simulink model "Inverter_32Vrms_StaticFreq_Fixed"  (R2025b)
settings: Solver=FixedStepDiscrete  StartTime=0.0  StopTime=0.35  FixedStep=SPWM_Ts  RelTol=1e-3
InitFcn:
  | evalin(get_param('Inverter_32Vrms_StaticFreq_Fixed','ModelWorkspace'),'assert(isscalar(SPWM_f1) && isfinite(SPWM_f1) && SPWM_f1>=20 && SPWM_f1<=100, ''SPWM_f1 must be 20 to 100 Hz.''); CL_N=round(1/(SPWM_f1*CL_Ts)); CL_AA_a=exp(-2*pi*CL_faa*SPWM_Ts); CL_AAComp=((1-CL_AA_a)^2+2*CL_AA_a*(1-cos(2*pi*SPWM_f1*SPWM_Ts)))/(1-CL_AA_a)^2;');
model workspace (MAT data in the model file):
  CL_AAComp = 1.00999999872
  CL_AA_a = 0.998744152176
  CL_Kaw = 20
  CL_Ki = 1.2
  CL_Kp = 0.02
  CL_N = 100
  CL_Ts = 0.0001
  CL_Vref = 32
  CL_faa = 1000
  CL_fp = 50
  CL_mff = 0.95
  CL_mmax = 1
  SPWM_Ndead = 10
  SPWM_Tdead = 2e-06
  SPWM_Ts = 2e-07
  SPWM_Vgate = 10
  SPWM_f1 = 100
  SPWM_fs = 20000
  SPWM_m = 0.8
undefined symbols (not defined in the file): DiscIntNeverNeededParam
libraries: fl_lib x19, ee_lib x13, nesl_utility x13
settings Model: Creator=liuhaobo  LastModifiedBy=liuhaobo

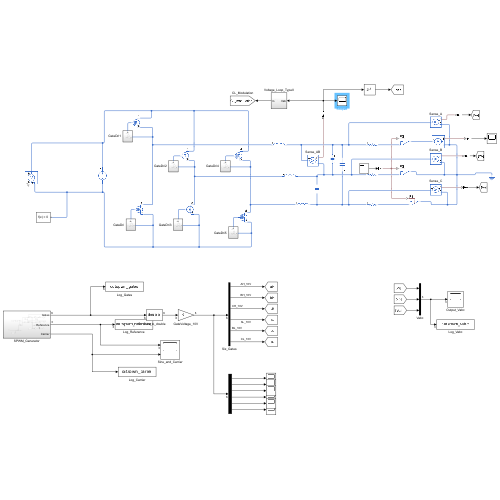
[thumbnail: Simulink's stored preview of the top-level diagram]
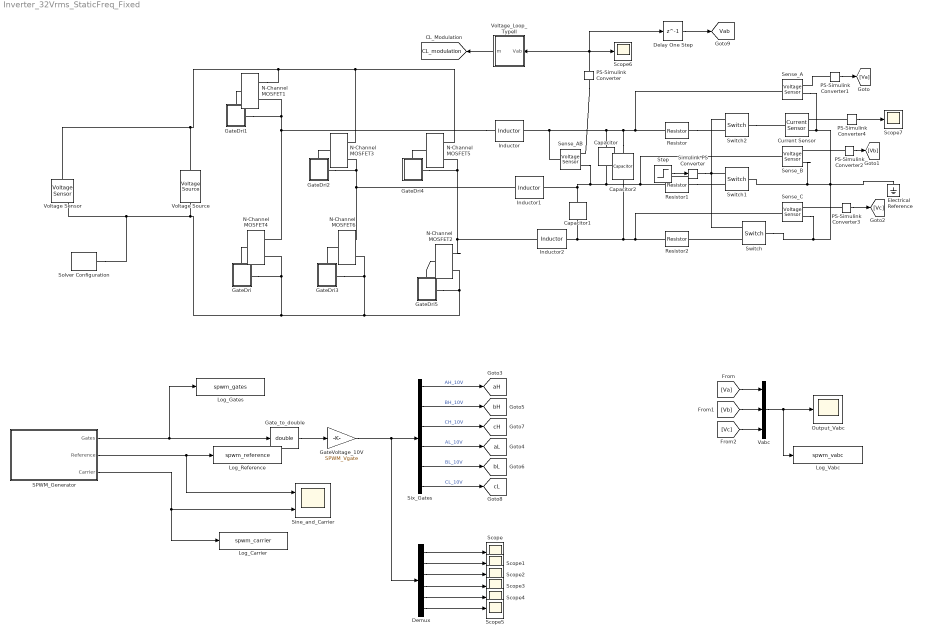
== system Inverter_32Vrms_StaticFreq_Fixed ==
  Capacitor : ee_lib/Passive/Capacitor  cap_option=ee.enum.passive.capacitor.capOption.const  c=2 uF  Cvec=[1e-05, 1e-06] F  Vvec=[0, 10] V  CV_table_symmetry=ee.enum.passive.capacitor.tableSymmetry.yes  f_vec=[1, 10] kHz  DFext_vec=[.8, 1.2]  enable_C_tol=ee.enum.toleranceApplication.none  averaging_period=0 s  C_tol=5  tol_distribution=ee.enum.toleranceDistribution.uniform  nSigma=4  r=0 Ohm  g=0 1/Ohm  enable_operating_limits=ee.enum.enable.no  operating_limit_action=ee.enum.passive.reportOpLim.warn  max_working_voltage_range=[-25, 25] V  power_rating=1 W  maxTemperature=85 degC  thermalEnable=false  thermalMass=1 J/K  i_specify=off  i_priority=None  i=0 A  i_nominal_specify=off  i_nominal_value=1  i_nominal_unit=A  v_specify=off  v_priority=None  v=0 V  v_nominal_specify=off  v_nominal_value=1  v_nominal_unit=V  vc_specify=off  vc_priority=High  vc=0 V  vc_nominal_specify=off  vc_nominal_value=1  vc_nominal_unit=V  T_specify=off  T_priority=None  T=298.15 K  T_nominal_specify=off  T_nominal_value=1  T_nominal_unit=K
  Capacitor1 : ee_lib/Passive/Capacitor  cap_option=ee.enum.passive.capacitor.capOption.const  c=2 uF  Cvec=[1e-05, 1e-06] F  Vvec=[0, 10] V  CV_table_symmetry=ee.enum.passive.capacitor.tableSymmetry.yes  f_vec=[1, 10] kHz  DFext_vec=[.8, 1.2]  enable_C_tol=ee.enum.toleranceApplication.none  averaging_period=0 s  C_tol=5  tol_distribution=ee.enum.toleranceDistribution.uniform  nSigma=4  r=0 Ohm  g=0 1/Ohm  enable_operating_limits=ee.enum.enable.no  operating_limit_action=ee.enum.passive.reportOpLim.warn  max_working_voltage_range=[-25, 25] V  power_rating=1 W  maxTemperature=85 degC  thermalEnable=false  thermalMass=1 J/K  i_specify=off  i_priority=None  i=0 A  i_nominal_specify=off  i_nominal_value=1  i_nominal_unit=A  v_specify=off  v_priority=None  v=0 V  v_nominal_specify=off  v_nominal_value=1  v_nominal_unit=V  vc_specify=off  vc_priority=High  vc=0 V  vc_nominal_specify=off  vc_nominal_value=1  vc_nominal_unit=V  T_specify=off  T_priority=None  T=298.15 K  T_nominal_specify=off  T_nominal_value=1  T_nominal_unit=K
  Capacitor2 : ee_lib/Passive/Capacitor  cap_option=ee.enum.passive.capacitor.capOption.const  c=2 uF  Cvec=[1e-05, 1e-06] F  Vvec=[0, 10] V  CV_table_symmetry=ee.enum.passive.capacitor.tableSymmetry.yes  f_vec=[1, 10] kHz  DFext_vec=[.8, 1.2]  enable_C_tol=ee.enum.toleranceApplication.none  averaging_period=0 s  C_tol=5  tol_distribution=ee.enum.toleranceDistribution.uniform  nSigma=4  r=0 Ohm  g=0 1/Ohm  enable_operating_limits=ee.enum.enable.no  operating_limit_action=ee.enum.passive.reportOpLim.warn  max_working_voltage_range=[-25, 25] V  power_rating=1 W  maxTemperature=85 degC  thermalEnable=false  thermalMass=1 J/K  i_specify=off  i_priority=None  i=0 A  i_nominal_specify=off  i_nominal_value=1  i_nominal_unit=A  v_specify=off  v_priority=None  v=0 V  v_nominal_specify=off  v_nominal_value=1  v_nominal_unit=V  vc_specify=off  vc_priority=High  vc=0 V  vc_nominal_specify=off  vc_nominal_value=1  vc_nominal_unit=V  T_specify=off  T_priority=None  T=298.15 K  T_nominal_specify=off  T_nominal_value=1  T_nominal_unit=K
  Current Sensor : fl_lib/Electrical/Electrical Sensors/Current Sensor
  Delay One Step : Delay  DelayLength=1
  Demux : Demux  Outputs=6
  Electrical Reference : fl_lib/Electrical/Electrical Elements/Electrical Reference
  GateDri : Subsystem
      settings: PortSchema="{\"entries\":[{\"content\":{\"sides\":[{\"content\":{\"connectorIds\":[\"LConn1\"]},\"type\":\"ConnectorPlacement.EquallySpacedRectSide\",\"uuid\":\"5ec2b66a-2e5f-4a29-ad7d-11e5a28469f4\"},{\"content\":{\"side\":\"RIGHT\"},\"type\":\"ConnectorPlacement.EquallySpacedRectSide\",\"uuid\":\"968cf12b-ade8-46ac-9f94-1e8ea2f3f677\"},{\"content\":{\"side\":\"TOP\"},\"type\":\"ConnectorPlacement.EquallySpacedRectSide\",\"uuid\":\"41030f6a-5ac0-4230-aa4b-0c03378f97d6\"},{\"content\":{\"connectorIds\":[\"RConn1\"],\"side\":\"BOTTOM\"},\"type\":\"ConnectorPlacement.EquallySpacedRectSide\",\"uuid\":\"8f964c8e-6f21-4ad0-8f7c-edbb0b22c660\"}]},\"type\":\"ConnectorPlacement.EquallySpacedConnector\",\"uuid\":\"dccfb76b-3882-476d-8e51-da801e2932e6\"}],\"packageUris\":[\"http://schema.mathworks.com/mf0/Connector/R2020b\"],\"version\":\"1.0\"}"
  GateDri1 : Subsystem
      settings: PortSchema="{\"entries\":[{\"content\":{\"sides\":[{\"content\":{\"connectorIds\":[\"LConn1\"]},\"type\":\"ConnectorPlacement.EquallySpacedRectSide\",\"uuid\":\"5ec2b66a-2e5f-4a29-ad7d-11e5a28469f4\"},{\"content\":{\"side\":\"RIGHT\"},\"type\":\"ConnectorPlacement.EquallySpacedRectSide\",\"uuid\":\"968cf12b-ade8-46ac-9f94-1e8ea2f3f677\"},{\"content\":{\"side\":\"TOP\"},\"type\":\"ConnectorPlacement.EquallySpacedRectSide\",\"uuid\":\"41030f6a-5ac0-4230-aa4b-0c03378f97d6\"},{\"content\":{\"connectorIds\":[\"RConn1\"],\"side\":\"BOTTOM\"},\"type\":\"ConnectorPlacement.EquallySpacedRectSide\",\"uuid\":\"8f964c8e-6f21-4ad0-8f7c-edbb0b22c660\"}]},\"type\":\"ConnectorPlacement.EquallySpacedConnector\",\"uuid\":\"dccfb76b-3882-476d-8e51-da801e2932e6\"}],\"packageUris\":[\"http://schema.mathworks.com/mf0/Connector/R2020b\"],\"version\":\"1.0\"}"
  GateDri2 : Subsystem
      settings: PortSchema="{\"entries\":[{\"content\":{\"sides\":[{\"content\":{\"connectorIds\":[\"LConn1\"]},\"type\":\"ConnectorPlacement.EquallySpacedRectSide\",\"uuid\":\"5ec2b66a-2e5f-4a29-ad7d-11e5a28469f4\"},{\"content\":{\"side\":\"RIGHT\"},\"type\":\"ConnectorPlacement.EquallySpacedRectSide\",\"uuid\":\"968cf12b-ade8-46ac-9f94-1e8ea2f3f677\"},{\"content\":{\"side\":\"TOP\"},\"type\":\"ConnectorPlacement.EquallySpacedRectSide\",\"uuid\":\"41030f6a-5ac0-4230-aa4b-0c03378f97d6\"},{\"content\":{\"connectorIds\":[\"RConn1\"],\"side\":\"BOTTOM\"},\"type\":\"ConnectorPlacement.EquallySpacedRectSide\",\"uuid\":\"8f964c8e-6f21-4ad0-8f7c-edbb0b22c660\"}]},\"type\":\"ConnectorPlacement.EquallySpacedConnector\",\"uuid\":\"dccfb76b-3882-476d-8e51-da801e2932e6\"}],\"packageUris\":[\"http://schema.mathworks.com/mf0/Connector/R2020b\"],\"version\":\"1.0\"}"
  GateDri3 : Subsystem
      settings: PortSchema="{\"entries\":[{\"content\":{\"sides\":[{\"content\":{\"connectorIds\":[\"LConn1\"]},\"type\":\"ConnectorPlacement.EquallySpacedRectSide\",\"uuid\":\"5ec2b66a-2e5f-4a29-ad7d-11e5a28469f4\"},{\"content\":{\"side\":\"RIGHT\"},\"type\":\"ConnectorPlacement.EquallySpacedRectSide\",\"uuid\":\"968cf12b-ade8-46ac-9f94-1e8ea2f3f677\"},{\"content\":{\"side\":\"TOP\"},\"type\":\"ConnectorPlacement.EquallySpacedRectSide\",\"uuid\":\"41030f6a-5ac0-4230-aa4b-0c03378f97d6\"},{\"content\":{\"connectorIds\":[\"RConn1\"],\"side\":\"BOTTOM\"},\"type\":\"ConnectorPlacement.EquallySpacedRectSide\",\"uuid\":\"8f964c8e-6f21-4ad0-8f7c-edbb0b22c660\"}]},\"type\":\"ConnectorPlacement.EquallySpacedConnector\",\"uuid\":\"dccfb76b-3882-476d-8e51-da801e2932e6\"}],\"packageUris\":[\"http://schema.mathworks.com/mf0/Connector/R2020b\"],\"version\":\"1.0\"}"
  GateDri4 : Subsystem
      settings: PortSchema="{\"entries\":[{\"content\":{\"sides\":[{\"content\":{\"connectorIds\":[\"LConn1\"]},\"type\":\"ConnectorPlacement.EquallySpacedRectSide\",\"uuid\":\"5ec2b66a-2e5f-4a29-ad7d-11e5a28469f4\"},{\"content\":{\"side\":\"RIGHT\"},\"type\":\"ConnectorPlacement.EquallySpacedRectSide\",\"uuid\":\"968cf12b-ade8-46ac-9f94-1e8ea2f3f677\"},{\"content\":{\"side\":\"TOP\"},\"type\":\"ConnectorPlacement.EquallySpacedRectSide\",\"uuid\":\"41030f6a-5ac0-4230-aa4b-0c03378f97d6\"},{\"content\":{\"connectorIds\":[\"RConn1\"],\"side\":\"BOTTOM\"},\"type\":\"ConnectorPlacement.EquallySpacedRectSide\",\"uuid\":\"8f964c8e-6f21-4ad0-8f7c-edbb0b22c660\"}]},\"type\":\"ConnectorPlacement.EquallySpacedConnector\",\"uuid\":\"dccfb76b-3882-476d-8e51-da801e2932e6\"}],\"packageUris\":[\"http://schema.mathworks.com/mf0/Connector/R2020b\"],\"version\":\"1.0\"}"
  GateDri5 : Subsystem
      settings: PortSchema="{\"entries\":[{\"content\":{\"sides\":[{\"content\":{\"connectorIds\":[\"LConn1\"]},\"type\":\"ConnectorPlacement.EquallySpacedRectSide\",\"uuid\":\"5ec2b66a-2e5f-4a29-ad7d-11e5a28469f4\"},{\"content\":{\"side\":\"RIGHT\"},\"type\":\"ConnectorPlacement.EquallySpacedRectSide\",\"uuid\":\"968cf12b-ade8-46ac-9f94-1e8ea2f3f677\"},{\"content\":{\"side\":\"TOP\"},\"type\":\"ConnectorPlacement.EquallySpacedRectSide\",\"uuid\":\"41030f6a-5ac0-4230-aa4b-0c03378f97d6\"},{\"content\":{\"connectorIds\":[\"RConn1\"],\"side\":\"BOTTOM\"},\"type\":\"ConnectorPlacement.EquallySpacedRectSide\",\"uuid\":\"8f964c8e-6f21-4ad0-8f7c-edbb0b22c660\"}]},\"type\":\"ConnectorPlacement.EquallySpacedConnector\",\"uuid\":\"dccfb76b-3882-476d-8e51-da801e2932e6\"}],\"packageUris\":[\"http://schema.mathworks.com/mf0/Connector/R2020b\"],\"version\":\"1.0\"}"
  GateVoltage_10V : Gain  Gain=SPWM_Vgate
  Gate_to_double : DataTypeConversion  OutDataTypeStr=double  SaturateOnIntegerOverflow=off  RndMeth=Floor
  Inductor : ee_lib/Passive/Inductor  l=680 uH  enable_L_tol=ee.enum.toleranceApplication.none  L_tol=20  tol_distribution=ee.enum.toleranceDistribution.uniform  nSigma=4  r=0 Ohm  g=1e-9 1/Ohm  enable_operating_limits=ee.enum.enable.no  operating_limit_action=ee.enum.passive.reportOpLim.warn  max_working_current=1 A  power_rating=1 W  i_L_specify=off  i_L_priority=High  i_L=0 A  i_L_nominal_specify=off  i_L_nominal_value=1  i_L_nominal_unit=A
  Inductor1 : ee_lib/Passive/Inductor  l=680 uH  enable_L_tol=ee.enum.toleranceApplication.none  L_tol=20  tol_distribution=ee.enum.toleranceDistribution.uniform  nSigma=4  r=0 Ohm  g=1e-9 1/Ohm  enable_operating_limits=ee.enum.enable.no  operating_limit_action=ee.enum.passive.reportOpLim.warn  max_working_current=1 A  power_rating=1 W  i_L_specify=off  i_L_priority=High  i_L=0 A  i_L_nominal_specify=off  i_L_nominal_value=1  i_L_nominal_unit=A
  Inductor2 : ee_lib/Passive/Inductor  l=680 uH  enable_L_tol=ee.enum.toleranceApplication.none  L_tol=20  tol_distribution=ee.enum.toleranceDistribution.uniform  nSigma=4  r=0 Ohm  g=1e-9 1/Ohm  enable_operating_limits=ee.enum.enable.no  operating_limit_action=ee.enum.passive.reportOpLim.warn  max_working_current=1 A  power_rating=1 W  i_L_specify=off  i_L_priority=High  i_L=0 A  i_L_nominal_specify=off  i_L_nominal_value=1  i_L_nominal_unit=A
  Log_Carrier : ToWorkspace  VariableName=spwm_carrier  SaveFormat=Timeseries  SampleTime=-1
  Log_Gates : ToWorkspace  VariableName=spwm_gates  SaveFormat=Timeseries  SampleTime=-1
  Log_Reference : ToWorkspace  VariableName=spwm_reference  SaveFormat=Timeseries  SampleTime=-1
  Log_Vabc : ToWorkspace  VariableName=spwm_vabc  SaveFormat=Timeseries  SampleTime=-1
  N-Channel MOSFET{1..6} (6 alike) : ee_lib/Semiconductors & Converters/N-Channel MOSFET  paramTerminal=ee.enum.mosfet.numberOfTerminals.three  parameterization=ee.enum.mosfet.parameterization.datasheet  Beta=5.0 A/V^2  Rds=0.025 Ohm  Id=6.0 A  Vgs=10 V  Vth=1.7 V  Vth0=1.7 V  lam=0 1/V  gamma_vth=0.5 V^(1/2)  phib=0.5 V  Vth1=1.9071 V  Vbs1=-1 V  Vth2=2.066 V  Vbs2=-2 V  Tmeas=25 degC  Vgs_vec=[-1, -.5, 2, 3, 4, 5] V  Vds_vec=[0, 2, 4, 8, 12, 16, 20] V  Vbs_vec=[0, -4, -6, -12] V  T_vec=[25, 125] degC  Vth_vec=[.4, 1.2, 1.4, 1.45] V  Vth_mat=[.4, .35; 1.2, 1.15; 1.4, 1.35; 1.45, 1.4] V  Ids_mat=[0, 0, 0, 0, 0, 0, 0; 0, 0, 0, 0, 0, 0, 0; 0, .003, .0038, .0043, .0046, .0048, .0049; 0, .0055, .008, .009, .0095, .01, .0101; 0, .0115, .016, .018, .019, .0195, .02; 0, .0152, .0225, .0265, .028, .0295, .03] A  Ids_mat0=[0, 0, 0, 0, 0, 0, 0; 0, 0, 0, 0, 0, 0, 0; 0, .003, .0038, .0043, .0046, .0048, .0049; 0, .0055, .008, .009, .0095, .01, .0101; 0, .0115, .016, .018, .019, .0195, .02; 0, .0152, .0225, .0265, .028, .0295, .03] A  Ids_mat_3D=zeros(6, 7, 2) A  Ids_mat_3D0=zeros(6, 7, 2) A  IV_table_symmetry=ee.enum.mosfet.symmetricNIV.no  RS=0.0001 Ohm  RD=0.01 Ohm  RB=0.001 Ohm  LeadRs=0 Ohm  LeadRd=0 Ohm  LeadRg=0 Ohm  LeadRb=0 Ohm  LS=0 nH  LD=0 nH  LG=0 nH  LB=0 nH  C_param=ee.enum.mosfet.capacitanceParam.fixedciss  C_GS=270 pF  C_GD=80 pF  C_GB=0 pF  C_DS=0 pF  C_iss=350 pF  C_rss=80 pF  C_oss=0 pF  C_iss_vec=[720, 700, 590, 470, 390, 310] pF  C_rss_vec=[450, 400, 300, 190, 95, 55] pF  C_oss_vec=[900, 810, 690, 420, 270, 170] pF  C_GS_vec=[270, 300, 290, 280, 295, 255] pF  C_GD_vec=[450, 400, 300, 190, 95, 55] pF  C_GB_vec=[270, 300, 290, 280, 295, 255] pF  C_Vgs_vec=0 V  C_DS_vec=[450, 410, 390, 230, 175, 115] pF  C_Vds_vec=[.1, .3, 1, 3, 10, 30] V  V_GS_for_cap_data=0 V  charge_linearity_param=ee.enum.mosfet.cgdLinearity.constant  C_OX=200 pF  V_C_OX=-0.5 V  charge_linearity_param_vgb=ee.enum.mosfet.cgbLinearity.instantly  charge_linearity_param_with_vgb=ee.enum.mosfet.cgbLinearityWithSeparateCgb.instantly  Di_param=ee.enum.mosfet.diodeParam.exponential  IsDiode=1e-12 A  Vbi=0.6 V  n=1  Cj0Diode=0 pF  TT=50e-9 s  Tmeas_dio=25 degC  TableTypeNoT=ee.enum.mosfet.tableType.IfMat  TableType=ee.enum.diode.tableType.IfMat  IfVec=[.07, .12, .19, 1.75, 4.24, 7.32, 11.2] A  IfMat=[.07, .12, .19, 1.75, 4.24, 7.32, 11.2; .16, .3, .72, 2.14, 4.02, 6.35, 9.12] A  VfVecV=[.9, 1.15, 1.25, 1.5, 1.75, 2.17, 2.6, 2.85] V  VfMatV=[.9, 1.15, 1.25, 1.5, 1.75, 2.17, 2.6, 2.85; .58, .68, .75, 1.1, 1.38, 1.77, 2.27, 2.7] V  TjVec=[25, 125] degC  VfVec=[.5, .7, .9, 1.3, 1.7, 2.1, 2.5] V  IfVecV=[.1, .2, .5, 1, 2, 4, 7, 10] A  diode_Goff=1e-12 1/Ohm  prmDatasheet=ee.enum.temperatureParameterization.simulation  prmEquCoeff=ee.enum.temperatureParameterization.none  dVth_dT=-6 mV/K  dVth0_dT=-6 mV/K  Rds_T2=0.037 Ohm  BEXDatasheet=-1.5  BEXEquCoeff=-1.5  etaisDatasheet=3  etaisEquCoeff=3  Tmeas2=125 degC  etaisTabulated=3  TdeviceDatasheet=25 degC  TdeviceEquCoeff=25 degC  TdeviceTabulated=25 degC  i_g_specify=off  i_g_priority=None  i_g=0 A  i_g_nominal_specify=off  i_g_nominal_value=1  i_g_nominal_unit=A  i_d_specify=off  i_d_priority=None  i_d=0 A  i_d_nominal_specify=off  i_d_nominal_value=1  i_d_nominal_unit=A  i_b_specify=off  i_b_priority=None  i_b=0 A  i_b_nominal_specify=off  i_b_nominal_value=1  i_b_nominal_unit=A  voltage_gs_specify=off  voltage_gs_priority=None  voltage_gs=0 V  voltage_gs_nominal_specify=off  voltage_gs_nominal_value=1  voltage_gs_nominal_unit=V  voltage_ds_specify=off  voltage_ds_priority=None  voltage_ds=0 V  voltage_ds_nominal_specify=off  voltage_ds_nominal_value=1  voltage_ds_nominal_unit=V  voltage_bs_specify=off  voltage_bs_priority=None  voltage_bs=0 V  voltage_bs_nominal_specify=off  voltage_bs_nominal_value=1  voltage_bs_nominal_unit=V  v_Cgs_specify=off  v_Cgs_priority=High  v_Cgs=0 V  v_Cgs_nominal_specify=off  v_Cgs_nominal_value=1  v_Cgs_nominal_unit=V  v_Cds_specify=off  v_Cds_priority=High  v_Cds=0 V  v_Cds_nominal_specify=off  v_Cds_nominal_value=1  v_Cds_nominal_unit=V  v_Cbs_specify=off  v_Cbs_priority=High  v_Cbs=0 V  v_Cbs_nominal_specify=off  v_Cbs_nominal_value=1  v_Cbs_nominal_unit=V  thermal_network_parameterization=ee.enum.thermalNetworkTopology.junctionCase  Rth=[0, 10] K/W  Rth_Cauer=[1, 3, 10] K/W  Rth_Foster=[.08, .14, .22, .16] K/W  thermal_mass_parameterization=ee.enum.thermalNetwork.timeconstant  thermal_mass=[0, 1] J/K  thermal_mass_Cauer=[.1, .3, 1] J/K  thermal_mass_Foster=[.001, .005, .05, .5] J/K  thermal_time_constant=[0, 10] s  thermal_time_constant_Cauer=[1, 3, 10] s  thermal_time_constant_Foster=[7e-05, .0007, .01, .08] s  thermal_mass_initial_temperatures=[25, 25] degC  thermal_mass_initial_temperatures_Cauer=[25, 25, 25] degC  Tvec_initial_Foster=[25, 25, 25, 25] degC  betaref=18 A/V^2  Vfbref=-1.1 V  gamma=3.5 V^(1/2)  phib2ref=1 V  thesatref=0.4 1/V  alpha=0  Vp=5e-2 V  thesrref=0 1/V  m=8  Tref=25 degC  Rsref=2e-3 Ohm  Rdref=0.17 Ohm  Rgref=8.4 Ohm  Rbref=2e-3 Ohm  Cox=1500 pF  Cgso=100 pF  Cgdo=14 pF  Isref=5.2e-13 A  Cj0=480 pF  Tprm=1  etabet=1.3  Stvfb=5e-4 V/K  Stphib=-8.5e-4 V/K  etasat=1.04  etasr=0.65  etar=0.95  etais=3  Tsim=25 degC  Ig_specify=off  Ig_priority=None  Ig=0 A  Ig_nominal_specify=off  Ig_nominal_value=1  Ig_nominal_unit=nA  Ids_specify=off  Ids_priority=None  Ids=0 A  Ids_nominal_specify=off  Ids_nominal_value=1  Ids_nominal_unit=A  Ib_specify=off  Ib_priority=None  Ib=0 A  Ib_nominal_specify=off  Ib_nominal_value=1  Ib_nominal_unit=uA  V_gs_specify=off  V_gs_priority=None  V_gs=0 V  V_gs_nominal_specify=off  V_gs_nominal_value=1  V_gs_nominal_unit=V  V_ds_specify=off  V_ds_priority=None  V_ds=0 V  V_ds_nominal_specify=off  V_ds_nominal_value=1  V_ds_nominal_unit=V  V_bs_specify=off  V_bs_priority=None  V_bs=0 V  V_bs_nominal_specify=off  V_bs_nominal_value=1  V_bs_nominal_unit=V  QGoverCox_specify=off  QGoverCox_priority=None  QGoverCox=0 V  QGoverCox_nominal_specify=off  QGoverCox_nominal_value=1  QGoverCox_nominal_unit=V  QDoverCox_specify=off  QDoverCox_priority=None  QDoverCox=0 V  QDoverCox_nominal_specify=off  QDoverCox_nominal_value=1  QDoverCox_nominal_unit=V  QBoverCox_specify=off  QBoverCox_priority=None  QBoverCox=0 V  QBoverCox_nominal_specify=off  QBoverCox_nominal_value=1  QBoverCox_nominal_unit=V  T0=[25, 25] degC  T0_Cauer=[25, 25, 25] degC
  Output_Vabc : Scope
      settings: TimeSpan=0.04  ActiveDisplayYMinimum=-63.585427203829283  ActiveDisplayYMaximum=65.9324966743516
  PS-Simulink Converter{,1..4} (5 alike) : nesl_utility/PS-Simulink Converter  PhysicalDomain=network_engine_domain  SubClassName=ps_output  LeftPortType=input  RightPortType=output  PseudoPeriodic=off  Frequencies=[]  VectorFormat=inherit  Unit=inherit  AffineConversion=off
  Resistor : fl_lib/Electrical/Electrical Elements/Resistor  R=10 Ohm  i_specify=off  i_priority=None  i=0 A  i_nominal_specify=off  i_nominal_value=1  i_nominal_unit=A  v_specify=off  v_priority=None  v=0 V  v_nominal_specify=off  v_nominal_value=1  v_nominal_unit=V
  Resistor1 : fl_lib/Electrical/Electrical Elements/Resistor  R=10 Ohm  i_specify=off  i_priority=None  i=0 A  i_nominal_specify=off  i_nominal_value=1  i_nominal_unit=A  v_specify=off  v_priority=None  v=0 V  v_nominal_specify=off  v_nominal_value=1  v_nominal_unit=V
  Resistor2 : fl_lib/Electrical/Electrical Elements/Resistor  R=10 Ohm  i_specify=off  i_priority=None  i=0 A  i_nominal_specify=off  i_nominal_value=1  i_nominal_unit=A  v_specify=off  v_priority=None  v=0 V  v_nominal_specify=off  v_nominal_value=1  v_nominal_unit=V
  SPWM_Generator : Subsystem
  Scope{,1..7} (8 alike) : Scope
      Scope settings: ActiveDisplayYMinimum=-1.2499999999999998  ActiveDisplayYMaximum=11.25
      Scope1 settings: DataLoggingVariableName=ScopeData2
      Scope2 settings: ActiveDisplayYMinimum=-2.5321191259765632  ActiveDisplayYMaximum=13.421400405273438  DataLoggingVariableName=ScopeData3
      Scope3 settings: DataLoggingVariableName=ScopeData4
      Scope4 settings: DataLoggingVariableName=ScopeData5
      Scope5 settings: DataLoggingVariableName=ScopeData6
      Scope6 settings: ActiveDisplayYMinimum=-37.5286202063157  ActiveDisplayYMaximum=54.00663525893075  DataLoggingVariableName=ScopeData7
      Scope7 settings: ActiveDisplayYMinimum=-0.81314889255588541  ActiveDisplayYMaximum=2.4755637669012946  DataLoggingVariableName=ScopeData8
  Sense_A : fl_lib/Electrical/Electrical Sensors/Voltage Sensor
  Sense_AB : fl_lib/Electrical/Electrical Sensors/Voltage Sensor
  Sense_B : fl_lib/Electrical/Electrical Sensors/Voltage Sensor
  Sense_C : fl_lib/Electrical/Electrical Sensors/Voltage Sensor
  Simulink-PS Converter : nesl_utility/Simulink-PS Converter  PhysicalDomain=network_engine_domain  SubClassName=ps_input  LeftPortType=input  RightPortType=output  PseudoPeriodic=off  Frequencies=[]  NoiseDistribution=none  NoiseParameters=[]  Unit=1  AffineConversion=off  FilteringAndDerivatives=provide  SimscapeFilterOrder=1  InputFilterTimeConstant=0.001  UdotUserProvided=0
  Sine_and_Carrier : Scope  NumInputPorts=2
      settings: TimeSpan=0.001  ActiveDisplayYMinimum=-0.65671925840887468  ActiveDisplayYMaximum=0.835711534861707
  Six_Gates : Demux  Outputs=6
  Solver Configuration : nesl_utility/Solver Configuration  PhysicalDomain=network_engine_domain  SubClassName=solver  LeftPortType=input  RightPortType=generic  Tones=[]  Harmonics=[]  SimulateNoise=off  Profile=off  UseLocalSampling=off  EnableSwitchedLinearOptims=on  FrequencyDomain=off  UseCCode=off  RelTol=0.001  AbsTol=0.001  MinStep=1e-09  ToWorkspace=off  RevertToSquareIcSolve=off  NumHomotopyIterations=100  PhasorMode=off  PhasorModeNumHarmonics=1  ConsistencySolver=NEWTON_XTOL_AFTER_FTOL  IndexReductionMethod=DerivativeReplacement  DoDC=off  ResidualTolerance=1e-09  ConsistencyTolSource=GLOBAL  ConsistencyAbsTol=0.001  ConsistencyRelTol=0.001  ConsistencyTolFactor=0.001  UseLocalSolver=on  LocalSolverChoice=NE_BACKWARD_EULER_ADVANCER  ResolveIndetEquations=on  FunctionEvalNumThread=1  LocalSolverSampleTime=SPWM_Ts  DoFixedCost=off  MaxNonlinIter=3  MaxModeIter=2  ComputeImpulses=off  ImpulseIterations=2  LinearAlgebra=auto  LinearAlgebraNumThread=0  EquationFormulation=NE_TIME_EF  DelaysMemoryBudget=1024  AutomaticFiltering=on  FilteringTimeConstant=0.001  PartitionStorageMethod=AS_NEEDED  PartitionMemoryBudget=1024  PartitionMethod=ROBUST  MultibodyUseLocalSolver=off  MultibodyLocalSolverChoice=ODE1  MultibodyLocalSolverSampleTime=0.001
  Step : Step  Time=0.15  Before=1  After=0  SampleTime=0
  Switch : fl_lib/Electrical/Electrical Elements/Switch  R_closed=0.01 Ohm  G_open=1e-8 1/Ohm  Threshold=0.5  i_specify=off  i_priority=None  i=0 A  i_nominal_specify=off  i_nominal_value=1  i_nominal_unit=A  v_specify=off  v_priority=None  v=0 V  v_nominal_specify=off  v_nominal_value=1  v_nominal_unit=V
  Switch1 : fl_lib/Electrical/Electrical Elements/Switch  R_closed=0.01 Ohm  G_open=1e-8 1/Ohm  Threshold=0.5  i_specify=off  i_priority=None  i=0 A  i_nominal_specify=off  i_nominal_value=1  i_nominal_unit=A  v_specify=off  v_priority=None  v=0 V  v_nominal_specify=off  v_nominal_value=1  v_nominal_unit=V
  Switch2 : fl_lib/Electrical/Electrical Elements/Switch  R_closed=0.01 Ohm  G_open=1e-8 1/Ohm  Threshold=0.5  i_specify=off  i_priority=None  i=0 A  i_nominal_specify=off  i_nominal_value=1  i_nominal_unit=A  v_specify=off  v_priority=None  v=0 V  v_nominal_specify=off  v_nominal_value=1  v_nominal_unit=V
  Vabc : Mux  Inputs=3
  Voltage Sensor : fl_lib/Electrical/Electrical Sensors/Voltage Sensor
  Voltage Source : ee_lib/Sources/Voltage Source  dc_voltage=60 V  ac_voltage=0 V  ac_shift=0 rad  ac_frequency=50 Hz  noise_mode=ee.enum.sources.noise.Disabled  PSD=0 V^2/Hz  sample_time=1e-3 s  repeatability=ee.enum.sources.repeatability.NotRepeatable  user_seed=0  auto_seed=3499211588  i_specify=off  i_priority=None  i=0 A  i_nominal_specify=off  i_nominal_value=1  i_nominal_unit=A  v_specify=off  v_priority=None  v=0 V  v_nominal_specify=off  v_nominal_value=1  v_nominal_unit=V
  Voltage_Loop_TypeII : Subsystem
  tag scope: CL_modulation=global, Vab=global, aH=global, aL=global, bH=global, bL=global, cH=global, cL=global
  wires:
  [Vc] -> Vabc/3
  [Vb] -> Vabc/2
  [Va] -> Vabc/1
  Vabc/1 -> Log_Vabc/1, Output_Vabc/1
  SPWM_Generator/3(Carrier) -> Sine_and_Carrier/2, Log_Carrier/1
  SPWM_Generator/2(Reference) -> Sine_and_Carrier/1, Log_Reference/1
  GateVoltage_10V/1 -> Demux/1, Six_Gates/1
  Gate_to_double/1 -> GateVoltage_10V/1
  SPWM_Generator/1(Gates) -> Log_Gates/1, Gate_to_double/1
  Six_Gates/1 -> [aH]  "AH_10V"
  Six_Gates/2 -> [bH]  "BH_10V"
  Six_Gates/3 -> [cH]  "CH_10V"
  Six_Gates/4 -> [aL]  "AL_10V"
  Six_Gates/5 -> [bL]  "BL_10V"
  Six_Gates/6 -> [cL]  "CL_10V"
  PS-Simulink Converter1/1 -> [Va]
  PS-Simulink Converter2/1 -> [Vb]
  PS-Simulink Converter3/1 -> [Vc]
  Demux/6 -> Scope5/1
  Demux/1 -> Scope/1
  Demux/2 -> Scope1/1
  Demux/3 -> Scope2/1
  Demux/4 -> Scope3/1
  Demux/5 -> Scope4/1
  Delay One Step/1 -> [Vab]
  Voltage_Loop_TypeII/1(m) -> [CL_modulation]
  PS-Simulink Converter/1 -> Delay One Step/1, Voltage_Loop_TypeII/1(Vab), Scope6/1
  Step/1 -> Simulink-PS Converter/1
  PS-Simulink Converter4/1 -> Scope7/1
  connections:
  Sense_C/RConn2 -- Switch/LConn1 -- Electrical Reference/LConn1 -- Sense_B/RConn2 -- Switch1/LConn1 -- Sense_A/RConn2 -- Current Sensor/RConn2
  Capacitor2/RConn1 -- Resistor2/LConn1 -- Sense_C/LConn1 -- Capacitor1/RConn1 -- Inductor2/RConn1
  Sense_B/LConn1 -- Resistor1/LConn1 -- Sense_AB/RConn2 -- Inductor1/RConn1 -- Capacitor1/LConn1 -- Capacitor/RConn1
  Capacitor2/LConn1 -- Resistor/LConn1 -- Sense_A/LConn1 -- Capacitor/LConn1 -- Sense_AB/LConn1 -- Inductor/RConn1
  GateDri3/RConn1 -- N-Channel MOSFET6/RConn2 -- N-Channel MOSFET2/RConn2 -- GateDri5/RConn1 -- N-Channel MOSFET4/RConn2 -- GateDri/RConn1 -- Voltage Source/RConn1 -- Solver Configuration/RConn1 -- Voltage Sensor/RConn2
  Voltage Sensor/LConn1 -- N-Channel MOSFET3/RConn1 -- N-Channel MOSFET5/RConn1 -- N-Channel MOSFET1/RConn1 -- Voltage Source/LConn1
  N-Channel MOSFET2/RConn1 -- GateDri4/RConn1 -- N-Channel MOSFET5/RConn2 -- Inductor2/LConn1
  N-Channel MOSFET6/RConn1 -- Inductor1/LConn1 -- GateDri2/RConn1 -- N-Channel MOSFET3/RConn2
  Inductor/LConn1 -- GateDri1/RConn1 -- N-Channel MOSFET1/RConn2 -- N-Channel MOSFET4/RConn1
  PS-Simulink Converter1/LConn1 -- Sense_A/RConn1
  PS-Simulink Converter2/LConn1 -- Sense_B/RConn1
  PS-Simulink Converter3/LConn1 -- Sense_C/RConn1
  GateDri/LConn1 -- N-Channel MOSFET4/LConn1
  GateDri1/LConn1 -- N-Channel MOSFET1/LConn1
  GateDri2/LConn1 -- N-Channel MOSFET3/LConn1
  GateDri3/LConn1 -- N-Channel MOSFET6/LConn1
  GateDri4/LConn1 -- N-Channel MOSFET5/LConn1
  GateDri5/LConn1 -- N-Channel MOSFET2/LConn1
  PS-Simulink Converter/LConn1 -- Sense_AB/RConn1
  Switch/RConn2 -- Resistor2/RConn1
  Resistor1/RConn1 -- Switch1/RConn2
  Resistor/RConn1 -- Switch2/RConn2
  Simulink-PS Converter/RConn1 -- Switch2/RConn1 -- Switch1/RConn1 -- Switch/RConn1
  Switch2/LConn1 -- Current Sensor/LConn1
  PS-Simulink Converter4/LConn1 -- Current Sensor/RConn1

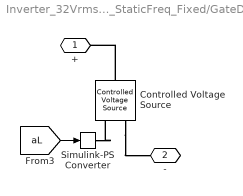
== system Inverter_32Vrms_StaticFreq_Fixed/GateDri ==
  Controlled Voltage Source : fl_lib/Electrical/Electrical Sources/Controlled Voltage Source
  Simulink-PS Converter : nesl_utility/Simulink-PS Converter  PhysicalDomain=network_engine_domain  SubClassName=ps_input  LeftPortType=input  RightPortType=output  PseudoPeriodic=off  Frequencies=[]  NoiseDistribution=none  NoiseParameters=[]  Unit=1  AffineConversion=off  FilteringAndDerivatives=provide  SimscapeFilterOrder=1  InputFilterTimeConstant=0.001  UdotUserProvided=0
  + : PMIOPort  Side=Left
  - : PMIOPort  Port=2  Side=Right
  wires:
  [aL] -> Simulink-PS Converter/1
  connections:
  Controlled Voltage Source/LConn1 -- +/RConn1
  Simulink-PS Converter/RConn1 -- Controlled Voltage Source/RConn1
  Controlled Voltage Source/RConn2 -- -/RConn1

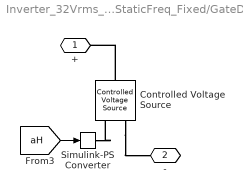
== system Inverter_32Vrms_StaticFreq_Fixed/GateDri1 ==
  Controlled Voltage Source : fl_lib/Electrical/Electrical Sources/Controlled Voltage Source
  Simulink-PS Converter : nesl_utility/Simulink-PS Converter  PhysicalDomain=network_engine_domain  SubClassName=ps_input  LeftPortType=input  RightPortType=output  PseudoPeriodic=off  Frequencies=[]  NoiseDistribution=none  NoiseParameters=[]  Unit=1  AffineConversion=off  FilteringAndDerivatives=provide  SimscapeFilterOrder=1  InputFilterTimeConstant=0.001  UdotUserProvided=0
  + : PMIOPort  Side=Left
  - : PMIOPort  Port=2  Side=Right
  wires:
  [aH] -> Simulink-PS Converter/1
  connections:
  Controlled Voltage Source/RConn2 -- -/RConn1
  Simulink-PS Converter/RConn1 -- Controlled Voltage Source/RConn1
  Controlled Voltage Source/LConn1 -- +/RConn1

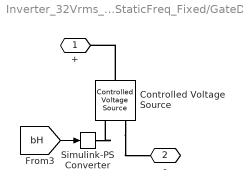
== system Inverter_32Vrms_StaticFreq_Fixed/GateDri2 ==
  Controlled Voltage Source : fl_lib/Electrical/Electrical Sources/Controlled Voltage Source
  Simulink-PS Converter : nesl_utility/Simulink-PS Converter  PhysicalDomain=network_engine_domain  SubClassName=ps_input  LeftPortType=input  RightPortType=output  PseudoPeriodic=off  Frequencies=[]  NoiseDistribution=none  NoiseParameters=[]  Unit=1  AffineConversion=off  FilteringAndDerivatives=provide  SimscapeFilterOrder=1  InputFilterTimeConstant=0.001  UdotUserProvided=0
  + : PMIOPort  Side=Left
  - : PMIOPort  Port=2  Side=Right
  wires:
  [bH] -> Simulink-PS Converter/1
  connections:
  Controlled Voltage Source/LConn1 -- +/RConn1
  Simulink-PS Converter/RConn1 -- Controlled Voltage Source/RConn1
  Controlled Voltage Source/RConn2 -- -/RConn1

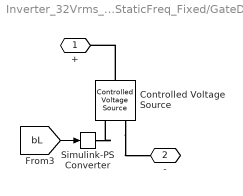
== system Inverter_32Vrms_StaticFreq_Fixed/GateDri3 ==
  Controlled Voltage Source : fl_lib/Electrical/Electrical Sources/Controlled Voltage Source
  Simulink-PS Converter : nesl_utility/Simulink-PS Converter  PhysicalDomain=network_engine_domain  SubClassName=ps_input  LeftPortType=input  RightPortType=output  PseudoPeriodic=off  Frequencies=[]  NoiseDistribution=none  NoiseParameters=[]  Unit=1  AffineConversion=off  FilteringAndDerivatives=provide  SimscapeFilterOrder=1  InputFilterTimeConstant=0.001  UdotUserProvided=0
  + : PMIOPort  Side=Left
  - : PMIOPort  Port=2  Side=Right
  wires:
  [bL] -> Simulink-PS Converter/1
  connections:
  Controlled Voltage Source/RConn2 -- -/RConn1
  Simulink-PS Converter/RConn1 -- Controlled Voltage Source/RConn1
  Controlled Voltage Source/LConn1 -- +/RConn1

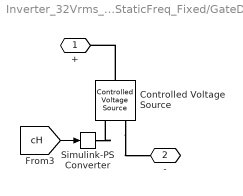
== system Inverter_32Vrms_StaticFreq_Fixed/GateDri4 ==
  Controlled Voltage Source : fl_lib/Electrical/Electrical Sources/Controlled Voltage Source
  Simulink-PS Converter : nesl_utility/Simulink-PS Converter  PhysicalDomain=network_engine_domain  SubClassName=ps_input  LeftPortType=input  RightPortType=output  PseudoPeriodic=off  Frequencies=[]  NoiseDistribution=none  NoiseParameters=[]  Unit=1  AffineConversion=off  FilteringAndDerivatives=provide  SimscapeFilterOrder=1  InputFilterTimeConstant=0.001  UdotUserProvided=0
  + : PMIOPort  Side=Left
  - : PMIOPort  Port=2  Side=Right
  wires:
  [cH] -> Simulink-PS Converter/1
  connections:
  Controlled Voltage Source/RConn2 -- -/RConn1
  Simulink-PS Converter/RConn1 -- Controlled Voltage Source/RConn1
  Controlled Voltage Source/LConn1 -- +/RConn1

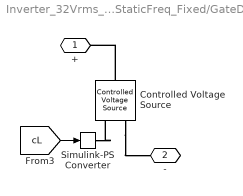
== system Inverter_32Vrms_StaticFreq_Fixed/GateDri5 ==
  Controlled Voltage Source : fl_lib/Electrical/Electrical Sources/Controlled Voltage Source
  Simulink-PS Converter : nesl_utility/Simulink-PS Converter  PhysicalDomain=network_engine_domain  SubClassName=ps_input  LeftPortType=input  RightPortType=output  PseudoPeriodic=off  Frequencies=[]  NoiseDistribution=none  NoiseParameters=[]  Unit=1  AffineConversion=off  FilteringAndDerivatives=provide  SimscapeFilterOrder=1  InputFilterTimeConstant=0.001  UdotUserProvided=0
  + : PMIOPort  Side=Left
  - : PMIOPort  Port=2  Side=Right
  wires:
  [cL] -> Simulink-PS Converter/1
  connections:
  Controlled Voltage Source/LConn1 -- +/RConn1
  Simulink-PS Converter/RConn1 -- Controlled Voltage Source/RConn1
  Controlled Voltage Source/RConn2 -- -/RConn1

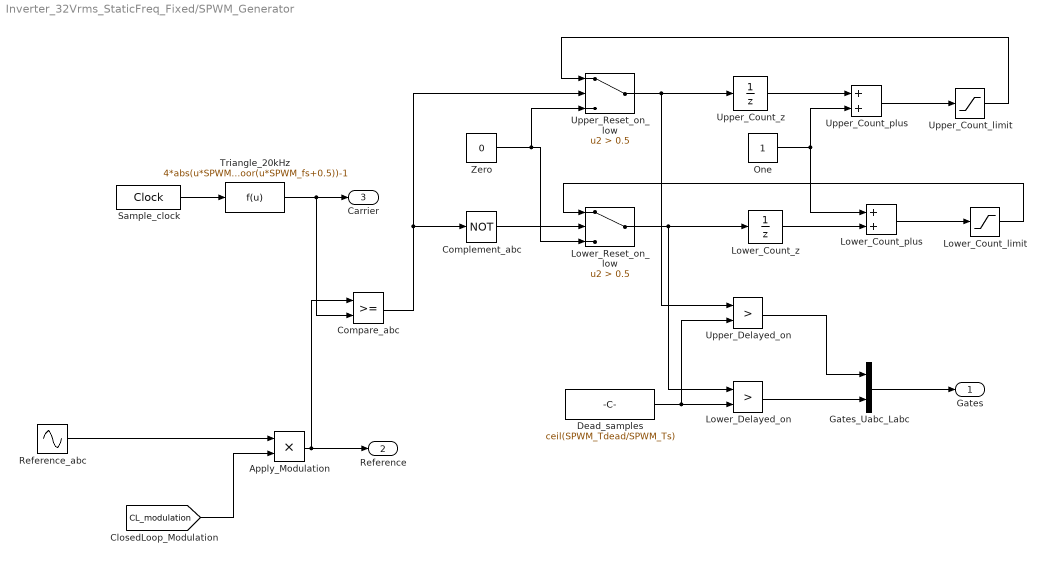
== system Inverter_32Vrms_StaticFreq_Fixed/SPWM_Generator ==
  Apply_Modulation : Product
  Compare_abc : RelationalOperator  OutDataTypeStr=boolean  RndMeth=Simplest  InputSameDT=off
  Complement_abc : Logic  Operator=NOT  Inputs=1  IconShape=distinctive  AllPortsSameDT=off  OutDataTypeStr=boolean
  Dead_samples : Constant  Value=ceil(SPWM_Tdead/SPWM_Ts)
  Gates_Uabc_Labc : Mux  Inputs=2
  Lower_Count_limit : Saturate  UpperLimit=ceil(SPWM_Tdead/SPWM_Ts)+1  LowerLimit=0
  Lower_Count_plus : Sum
  Lower_Count_z : UnitDelay  InitialCondition=[0 0 0]  SampleTime=SPWM_Ts  HasFrameUpgradeWarning=on
  Lower_Delayed_on : RelationalOperator  Operator=>  OutDataTypeStr=boolean  RndMeth=Simplest  InputSameDT=off
  Lower_Reset_on_low : Switch  Criteria=u2 > Threshold  Threshold=0.5  SaturateOnIntegerOverflow=off  InputSameDT=off
  One : Constant
  Reference_abc : Sin  Frequency=2*pi*SPWM_f1  Phase=[0 -2*pi/3 2*pi/3]  SampleTime=SPWM_Ts
  Sample_clock : DigitalClock  SampleTime=SPWM_Ts
  Triangle_20kHz : Fcn  Expr=4*abs(u*SPWM_fs-floor(u*SPWM_fs+0.5))-1
  Upper_Count_limit : Saturate  UpperLimit=ceil(SPWM_Tdead/SPWM_Ts)+1  LowerLimit=0
  Upper_Count_plus : Sum
  Upper_Count_z : UnitDelay  InitialCondition=[0 0 0]  SampleTime=SPWM_Ts  HasFrameUpgradeWarning=on
  Upper_Delayed_on : RelationalOperator  Operator=>  OutDataTypeStr=boolean  RndMeth=Simplest  InputSameDT=off
  Upper_Reset_on_low : Switch  Criteria=u2 > Threshold  Threshold=0.5  SaturateOnIntegerOverflow=off  InputSameDT=off
  Zero : Constant  Value=0
  Gates : Outport
  Reference : Outport  Port=2
  Carrier : Outport  Port=3
  wires:
  Gates_Uabc_Labc/1 -> Gates/1
  Lower_Delayed_on/1 -> Gates_Uabc_Labc/2
  Upper_Delayed_on/1 -> Gates_Uabc_Labc/1
  Lower_Reset_on_low/1 -> Lower_Count_z/1, Lower_Delayed_on/1
  Complement_abc/1 -> Lower_Reset_on_low/2
  Lower_Count_limit/1 -> Lower_Reset_on_low/1
  Lower_Count_plus/1 -> Lower_Count_limit/1
  Dead_samples/1 -> Upper_Delayed_on/2, Lower_Delayed_on/2
  Upper_Reset_on_low/1 -> Upper_Count_z/1, Upper_Delayed_on/1
  Zero/1 -> Upper_Reset_on_low/3, Lower_Reset_on_low/3
  Upper_Count_limit/1 -> Upper_Reset_on_low/1
  Upper_Count_plus/1 -> Upper_Count_limit/1
  One/1 -> Lower_Count_plus/1, Upper_Count_plus/2
  Upper_Count_z/1 -> Upper_Count_plus/1
  Sample_clock/1 -> Triangle_20kHz/1
  Lower_Count_z/1 -> Lower_Count_plus/2
  Apply_Modulation/1 -> Reference/1, Compare_abc/1
  [CL_modulation] -> Apply_Modulation/2
  Reference_abc/1 -> Apply_Modulation/1
  Triangle_20kHz/1 -> Carrier/1, Compare_abc/2
  Compare_abc/1 -> Complement_abc/1, Upper_Reset_on_low/2

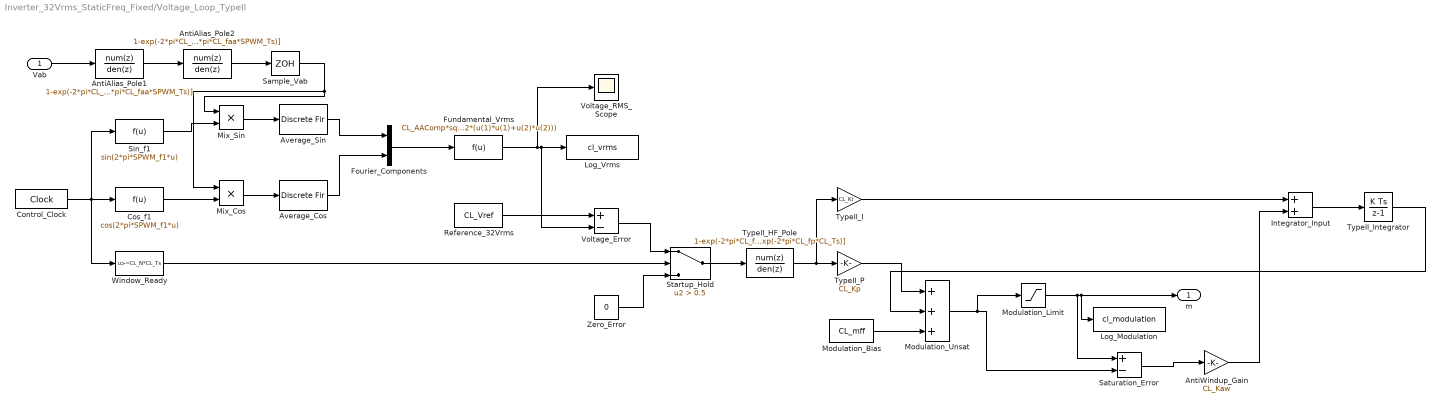
== system Inverter_32Vrms_StaticFreq_Fixed/Voltage_Loop_TypeII ==
  Vab : Inport
  AntiAlias_Pole1 : DiscreteTransferFcn  Numerator=1-exp(-2*pi*CL_faa*SPWM_Ts)  Denominator=[1 -exp(-2*pi*CL_faa*SPWM_Ts)]  SampleTime=SPWM_Ts
  AntiAlias_Pole2 : DiscreteTransferFcn  Numerator=1-exp(-2*pi*CL_faa*SPWM_Ts)  Denominator=[1 -exp(-2*pi*CL_faa*SPWM_Ts)]  SampleTime=SPWM_Ts
  AntiWindup_Gain : Gain  Gain=CL_Kaw
  Average_Cos : DiscreteFir  Coefficients=ones(1,CL_N)/CL_N  SampleTime=CL_Ts
  Average_Sin : DiscreteFir  Coefficients=ones(1,CL_N)/CL_N  SampleTime=CL_Ts
  Control_Clock : DigitalClock  SampleTime=CL_Ts
  Cos_f1 : Fcn  Expr=cos(2*pi*SPWM_f1*u)
  Fourier_Components : Mux  Inputs=2
  Fundamental_Vrms : Fcn  Expr=CL_AAComp*sqrt(2*(u(1)*u(1)+u(2)*u(2)))
  Integrator_Input : Sum
  Log_Modulation : ToWorkspace  VariableName=cl_modulation  SaveFormat=Timeseries  SampleTime=-1
  Log_Vrms : ToWorkspace  VariableName=cl_vrms  SaveFormat=Timeseries  SampleTime=-1
  Mix_Cos : Product
  Mix_Sin : Product
  Modulation_Bias : Constant  Value=CL_mff
  Modulation_Limit : Saturate  UpperLimit=CL_mmax  LowerLimit=0
  Modulation_Unsat : Sum  Inputs=+++
  Reference_32Vrms : Constant  Value=CL_Vref
  Sample_Vab : ZeroOrderHold  SampleTime=CL_Ts
  Saturation_Error : Sum  Inputs=+-
  Sin_f1 : Fcn  Expr=sin(2*pi*SPWM_f1*u)
  Startup_Hold : Switch  Criteria=u2 > Threshold  Threshold=0.5  SaturateOnIntegerOverflow=off  InputSameDT=off
  TypeII_HF_Pole : DiscreteTransferFcn  Numerator=1-exp(-2*pi*CL_fp*CL_Ts)  Denominator=[1 -exp(-2*pi*CL_fp*CL_Ts)]  SampleTime=CL_Ts
  TypeII_I : Gain  Gain=CL_Ki
  TypeII_Integrator : DiscreteIntegrator  SampleTime=CL_Ts  ICPrevOutput=DiscIntNeverNeededParam  ICPrevScaledInput=DiscIntNeverNeededParam
  TypeII_P : Gain  Gain=CL_Kp
  Voltage_Error : Sum  Inputs=+-
  Voltage_RMS_Scope : Scope
      settings: ActiveDisplayYMinimum=9.2272998775668817  ActiveDisplayYMaximum=44.022322654746958
  Window_Ready : Fcn  Expr=u>=CL_N*CL_Ts
  Zero_Error : Constant  Value=0
  m : Outport
  wires:
  Saturation_Error/1 -> AntiWindup_Gain/1
  Modulation_Limit/1 -> m/1, Log_Modulation/1, Saturation_Error/1
  Modulation_Unsat/1 -> Modulation_Limit/1, Saturation_Error/2
  Modulation_Bias/1 -> Modulation_Unsat/3
  TypeII_Integrator/1 -> Modulation_Unsat/2
  TypeII_P/1 -> Modulation_Unsat/1
  Integrator_Input/1 -> TypeII_Integrator/1
  AntiWindup_Gain/1 -> Integrator_Input/2
  TypeII_I/1 -> Integrator_Input/1
  TypeII_HF_Pole/1 -> TypeII_P/1, TypeII_I/1
  Startup_Hold/1 -> TypeII_HF_Pole/1
  Zero_Error/1 -> Startup_Hold/3
  Window_Ready/1 -> Startup_Hold/2
  Voltage_Error/1 -> Startup_Hold/1
  Reference_32Vrms/1 -> Voltage_Error/1
  Fundamental_Vrms/1 -> Voltage_Error/2, Log_Vrms/1, Voltage_RMS_Scope/1
  Fourier_Components/1 -> Fundamental_Vrms/1
  Average_Cos/1 -> Fourier_Components/2
  Average_Sin/1 -> Fourier_Components/1
  Mix_Cos/1 -> Average_Cos/1
  Mix_Sin/1 -> Average_Sin/1
  Cos_f1/1 -> Mix_Cos/2
  Sin_f1/1 -> Mix_Sin/2
  Control_Clock/1 -> Sin_f1/1, Cos_f1/1, Window_Ready/1
  AntiAlias_Pole2/1 -> Sample_Vab/1
  AntiAlias_Pole1/1 -> AntiAlias_Pole2/1
  Vab/1 -> AntiAlias_Pole1/1
  Sample_Vab/1 -> Mix_Sin/1, Mix_Cos/1
